simulink model "Exp3_Mamdani_FLC_DCmotor"  (R2025b)
settings: Solver=FixedStepDiscrete  StartTime=0  StopTime=8  FixedStep=0.01  RelTol=1e-3
undefined symbols (not defined in the file): Ad, Bd, Cd, Dd, DiscIntNeverNeededParam, Gde, Ge, Gu, Kd, Ki, Kp, openLoopGain, Ts, Vmax
libraries: fuzblock x1
settings Model: Creator=mithu  LastModifiedBy=mithu

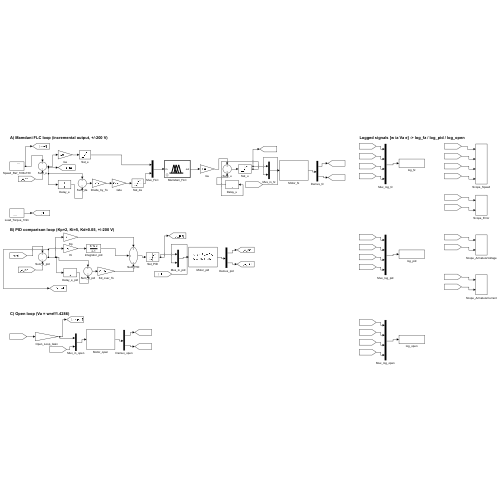
[thumbnail: Simulink's stored preview of the top-level diagram]
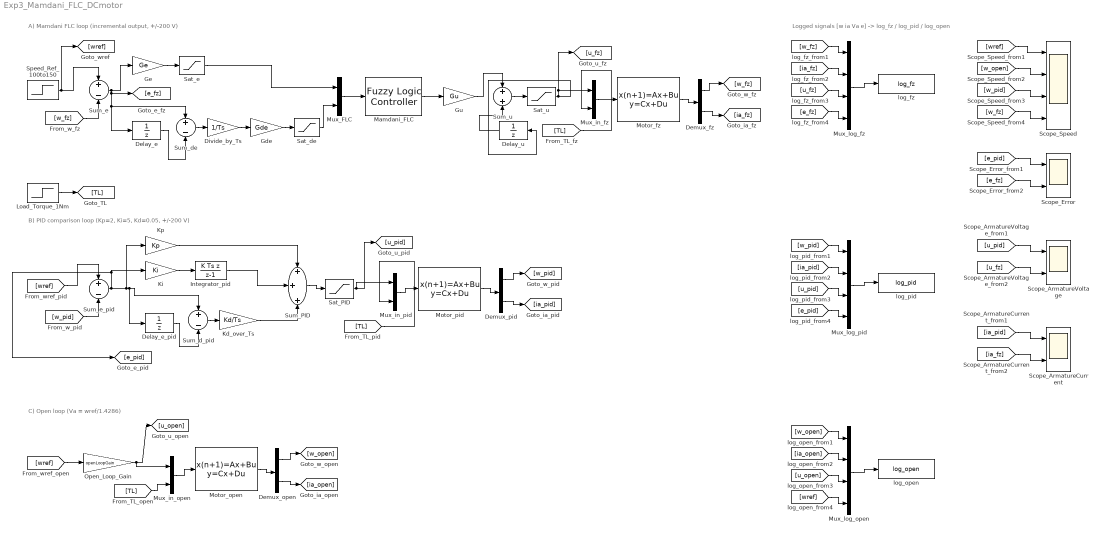
== system Exp3_Mamdani_FLC_DCmotor ==
  note: A) Mamdani FLC loop (incremental output, +/-200 V)
  note: B) PID comparison loop (Kp=2, Ki=5, Kd=0.05, +/-200 V)
  note: C) Open loop (Va = wref/1.4286)
  note: Logged signals [w ia Va e] -> log_fz / log_pid / log_open
  Delay_e : UnitDelay  SampleTime=Ts  HasFrameUpgradeWarning=on
  Delay_e_pid : UnitDelay  SampleTime=Ts  HasFrameUpgradeWarning=on
  Delay_u : UnitDelay  SampleTime=Ts  HasFrameUpgradeWarning=on
  Demux_fz : Demux  Outputs=2
  Demux_open : Demux  Outputs=2
  Demux_pid : Demux  Outputs=2
  Divide_by_Ts : Gain  Gain=1/Ts
  Gde : Gain  Gain=Gde
  Ge : Gain  Gain=Ge
  Gu : Gain  Gain=Gu
  Integrator_pid : DiscreteIntegrator  IntegratorMethod=Integration: Backward Euler  SampleTime=Ts  ICPrevOutput=DiscIntNeverNeededParam  ICPrevScaledInput=DiscIntNeverNeededParam
  Kd_over_Ts : Gain  Gain=Kd/Ts
  Ki : Gain  Gain=Ki
  Kp : Gain  Gain=Kp
  Load_Torque_1Nm : Step  Time=3  SampleTime=0
  Mamdani_FLC : fuzblock/Fuzzy Logic  Controller  FIS=fis  OutputSampleNumber=101  DataType=double  UseLookupTable=off  NumBreakpoints=10  FuzzifiedInputs=off  RuleFiringStrengths=off  RuleOutputs=off  AggregatedOutputs=off  SimulateUsing=Interpreted execution  OutOfRangeInputValueMessage=warning  NoRuleFiredMessage=warning  EmptyOutputFuzzySetMessage=warning
  Motor_fz : DiscreteStateSpace  A=Ad  B=Bd  C=Cd  D=Dd  SampleTime=Ts
  Motor_open : DiscreteStateSpace  A=Ad  B=Bd  C=Cd  D=Dd  SampleTime=Ts
  Motor_pid : DiscreteStateSpace  A=Ad  B=Bd  C=Cd  D=Dd  SampleTime=Ts
  Mux_FLC : Mux  Inputs=2
  Mux_in_fz : Mux  Inputs=2
  Mux_in_open : Mux  Inputs=2
  Mux_in_pid : Mux  Inputs=2
  Mux_log_fz : Mux
  Mux_log_open : Mux
  Mux_log_pid : Mux
  Open_Loop_Gain : Gain  Gain=openLoopGain
  Sat_PID : Saturate  UpperLimit=Vmax  LowerLimit=-Vmax
  Sat_de : Saturate  UpperLimit=1  LowerLimit=-1
  Sat_e : Saturate  UpperLimit=1  LowerLimit=-1
  Sat_u : Saturate  UpperLimit=Vmax  LowerLimit=-Vmax
  Scope_ArmatureCurrent : Scope  NumInputPorts=2
  Scope_ArmatureVoltage : Scope  NumInputPorts=2
  Scope_Error : Scope  NumInputPorts=2
  Scope_Speed : Scope  NumInputPorts=4
  Speed_Ref_100to150 : Step  Time=5  Before=100  After=150  SampleTime=0
  Sum_PID : Sum  Inputs=+++
  Sum_d_pid : Sum  Inputs=+-
  Sum_de : Sum  Inputs=+-
  Sum_e : Sum  Inputs=+-
  Sum_e_pid : Sum  Inputs=+-
  Sum_u : Sum
  log_fz : ToWorkspace  VariableName=log_fz  SaveFormat=Timeseries  SampleTime=Ts
  log_open : ToWorkspace  VariableName=log_open  SaveFormat=Timeseries  SampleTime=Ts
  log_pid : ToWorkspace  VariableName=log_pid  SaveFormat=Timeseries  SampleTime=Ts
  wires:
  Load_Torque_1Nm/1 -> [TL]
  Speed_Ref_100to150/1 -> Sum_e/1, [wref]
  [w_fz] -> Sum_e/2
  Sum_e/1 -> Delay_e/1, Sum_de/1, [e_fz], Ge/1
  Delay_e/1 -> Sum_de/2
  Ge/1 -> Sat_e/1
  Sat_e/1 -> Mux_FLC/1
  Sum_de/1 -> Divide_by_Ts/1
  Divide_by_Ts/1 -> Gde/1
  Gde/1 -> Sat_de/1
  Sat_de/1 -> Mux_FLC/2
  Mux_FLC/1 -> Mamdani_FLC/1
  Mamdani_FLC/1 -> Gu/1
  Gu/1 -> Sum_u/1
  Delay_u/1 -> Sum_u/2
  Sum_u/1 -> Sat_u/1
  Sat_u/1 -> [u_fz], Mux_in_fz/1, Delay_u/1
  [TL] -> Mux_in_fz/2
  Mux_in_fz/1 -> Motor_fz/1
  Motor_fz/1 -> Demux_fz/1
  Demux_fz/1 -> [w_fz]
  Demux_fz/2 -> [ia_fz]
  [wref] -> Sum_e_pid/1
  [w_pid] -> Sum_e_pid/2
  Sum_e_pid/1 -> Ki/1, [e_pid], Sum_d_pid/1, Delay_e_pid/1, Kp/1
  Delay_e_pid/1 -> Sum_d_pid/2
  Sum_d_pid/1 -> Kd_over_Ts/1
  Ki/1 -> Integrator_pid/1
  Kp/1 -> Sum_PID/1
  Integrator_pid/1 -> Sum_PID/2
  Kd_over_Ts/1 -> Sum_PID/3
  Sum_PID/1 -> Sat_PID/1
  Sat_PID/1 -> [u_pid], Mux_in_pid/1
  [TL] -> Mux_in_pid/2
  Mux_in_pid/1 -> Motor_pid/1
  Motor_pid/1 -> Demux_pid/1
  Demux_pid/1 -> [w_pid]
  Demux_pid/2 -> [ia_pid]
  [wref] -> Open_Loop_Gain/1
  Open_Loop_Gain/1 -> [u_open], Mux_in_open/1
  [TL] -> Mux_in_open/2
  Mux_in_open/1 -> Motor_open/1
  Motor_open/1 -> Demux_open/1
  Demux_open/1 -> [w_open]
  Demux_open/2 -> [ia_open]
  [w_fz] -> Mux_log_fz/1
  [ia_fz] -> Mux_log_fz/2
  [u_fz] -> Mux_log_fz/3
  [e_fz] -> Mux_log_fz/4
  Mux_log_fz/1 -> log_fz/1
  [w_pid] -> Mux_log_pid/1
  [ia_pid] -> Mux_log_pid/2
  [u_pid] -> Mux_log_pid/3
  [e_pid] -> Mux_log_pid/4
  Mux_log_pid/1 -> log_pid/1
  [w_open] -> Mux_log_open/1
  [ia_open] -> Mux_log_open/2
  [u_open] -> Mux_log_open/3
  [wref] -> Mux_log_open/4
  Mux_log_open/1 -> log_open/1
  [wref] -> Scope_Speed/1
  [w_open] -> Scope_Speed/2
  [w_pid] -> Scope_Speed/3
  [w_fz] -> Scope_Speed/4
  [e_pid] -> Scope_Error/1
  [e_fz] -> Scope_Error/2
  [u_pid] -> Scope_ArmatureVoltage/1
  [u_fz] -> Scope_ArmatureVoltage/2
  [ia_pid] -> Scope_ArmatureCurrent/1
  [ia_fz] -> Scope_ArmatureCurrent/2
